simulink model "mas508_lab2_exercise1"  (R2021b)
settings: Solver=FixedStepAuto  StartTime=0.0  StopTime=0.5  FixedStep=100e-6  RelTol=1e-3
values from neighbouring files (symbols this model uses):
  B = [0; 0; 1]    [L3d_e1_poleplacement.m]    (also in Lab5_solution.m = [0;1;0]; Lab6_example1.m = [2; -1]; Lab6_example2_3.m = [0 0 0 1/Jm]'; Lab6_extraproblem1.m)
  J = 0.00005    (= 5e-05)    [mas508_lab2_exercise1.m]    (also in mas508_lab2_exercise3_4.m = 0.011; mas508_problem2.m)
  L = 0.0002    [mas508_lab2_exercise1.m]    (also in mas508_problem2.m; mas508_problem3.m = [L1;L2])
  Psi = 0.04    [mas508_lab2_exercise1.m]
  R = diag([0.1])    [ExampleADP_main.m]    (also in mas508_lab2_exercise1.m = 1; mas508_problem2.m = 1)
settings Model: Creator=rtavares  LastModifiedBy=faisala
settings SolverCC: AlgebraicLoopSolver=TrustRegion
settings DebuggingCC: SFMachineParentedDataDiag=warning

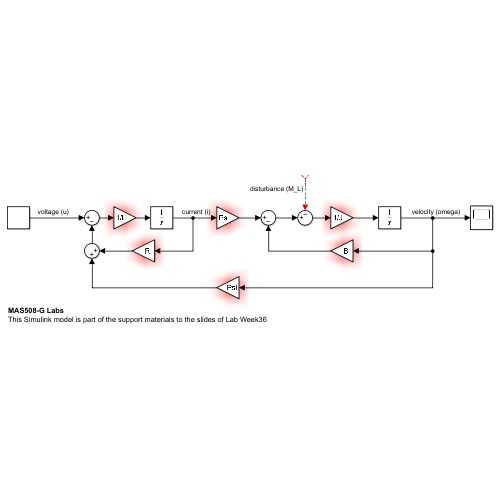
[thumbnail: Simulink's stored preview of the top-level diagram]
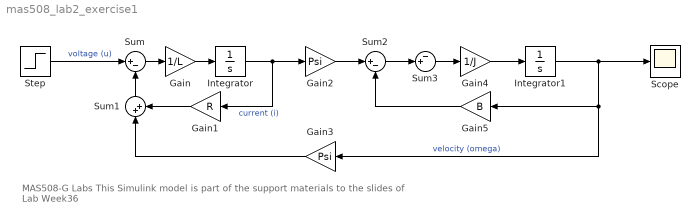
== system mas508_lab2_exercise1 ==
  note: MAS508-G Labs
      | This Simulink model is part of the support materials to the slides of Lab Week36
  Gain : Gain  Gain=1/L
  Gain1 : Gain  Gain=R
  Gain2 : Gain  Gain=Psi
  Gain3 : Gain  Gain=Psi
  Gain4 : Gain  Gain=1/J
  Gain5 : Gain  Gain=B
  Integrator : Integrator
  Integrator1 : Integrator
  Scope : Scope
  Step : Step  Time=0  SampleTime=0
  Sum : Sum  Inputs=|+-
  Sum1 : Sum  Inputs=|++
  Sum2 : Sum  Inputs=|+-
  Sum3 : Sum  Inputs=-+|
  wires:
  Gain/1 -> Integrator/1
  Integrator/1 -> Gain1/1, Gain2/1  "current (i)"
  Sum/1 -> Gain/1
  Sum1/1 -> Sum/2
  Gain1/1 -> Sum1/2
  Gain3/1 -> Sum1/1
  Gain2/1 -> Sum2/1
  Sum2/1 -> Sum3/2
  Gain4/1 -> Integrator1/1
  Sum3/1 -> Gain4/1
  Integrator1/1 -> Gain3/1, Gain5/1, Scope/1  "velocity (omega)"
  Gain5/1 -> Sum2/2
  Step/1 -> Sum/1  "voltage (u)"
  ? -> Sum3/1  "disturbance (M_L)"
